simulink library "cntrlPosNdi_lib"  (R2018b)
settings: Solver=VariableStepAuto  StartTime=0.0  StopTime=10.0  RelTol=1e-3
undefined symbols (not defined in the file or in its folder): DiscIntNeverNeededParam, psc
libraries: filters_lib x3, simulink x2, $bdroot x2, stick_lib x1
settings Model: Creator=Ybeyer  LastModifiedBy=yannic
settings SFSimCC: SimUseLocalCustomCode=off
settings RTWCC: RTWUseLocalCustomCode=off
settings CodeAppCC: StateflowObjectComments=on

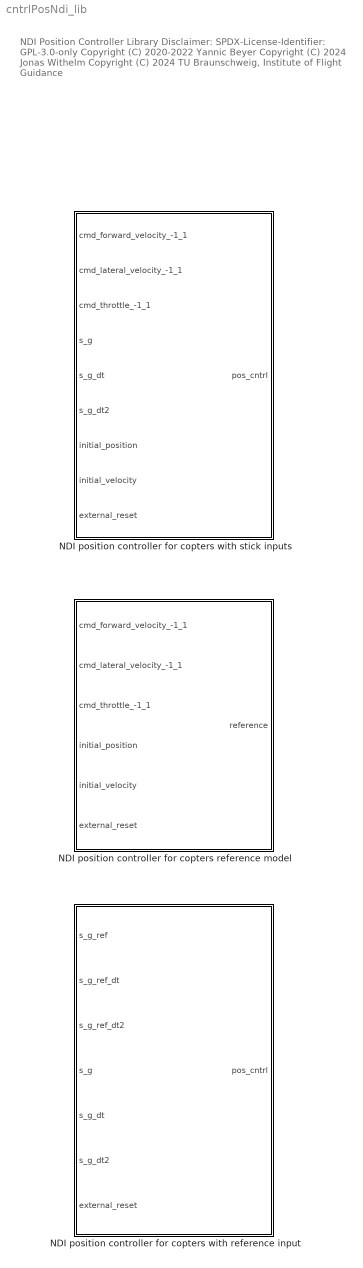
== system cntrlPosNdi_lib ==
  note: NDI Position Controller Library
      |
      | Disclaimer:
      | SPDX-License-Identifier: GPL-3.0-only
      |
      | Copyright (C) 2020-2022 Yannic Beyer
      | Copyright (C) 2024 Jonas Withelm
      | Copyright (C) 2024 TU Braunschweig, Institute of Flight Guidance
  NDI position controller for copters reference model : Subsystem  mask{psc=psc, is_enable_checked=off, states_when_enabling=held}
      mask prompts: psc "position controller parameters struct, see cntrlPosIndi_params_default"; is_enable_checked "Activate "Enabled Subsystem""; states_when_enabling "States when enabling:"
      mask init:
      | cntrlBlockInit(is_enable_checked,states_when_enabling);
      mask TypeOptions states_when_enabling: held | reset
      mask DialogControl DescGroupVar Prompt: NDI position controller for copters reference model
      mask DialogControl DescTextVar Prompt: The commanded velocity is filtered and reference signals are generated.
  NDI position controller for copters with reference input : Subsystem  mask{psc=psc, T_inner_loop=0.1, is_enable_checked=off, states_when_enabling=held, mask_expr_handling_config=default}
      mask prompts: psc "Position controller parameters struct, see cntrlPosIndi_params_default"; T_inner_loop "Inner loop time constant, in s"; is_enable_checked "Activate "Enabled Subsystem""; states_when_enabling "States when enabling:"
      mask init:
      | cntrlBlockInit(is_enable_checked,states_when_enabling);
      | 
      | maskExprHandling(gcbh, mask_expr_handling_config);
      mask TypeOptions states_when_enabling: held | reset
      mask TypeOptions mask_expr_handling_config: default | passthrough (tunable)
      mask DialogControl DescGroupVar Prompt: NDI position controller cascade with reference inputs
      mask DialogControl DescTextVar Prompt: The controller takes reference signals as input and the control error is converted into desired accerlations.
      mask DialogControl CodeGenerationSettings Prompt: Code Generation Settings
      mask DialogControl maskExprHandlingText Prompt: Mask expression handling
      mask DialogControl maskExprHandlingReadme Prompt: README
      mask DialogControl maskExprHandlingReadme Tooltip: https://github.com/iff-gsc/m-Utils/tree/main/simulink/mask_expression_handling/README.md
      mask DialogControl maskExprHandlingReadme Callback: web('https://github.com/iff-gsc/m-Utils/tree/main/simulink/mask_expression_handling/README.md','-browser')
  NDI position controller for copters with stick inputs : Subsystem  mask{psc=psc, T_inner_loop=0.1, is_enable_checked=off, states_when_enabling=held}
      mask prompts: psc "position controller parameters struct, see cntrlPosIndi_params_default"; T_inner_loop "inner loop time constant, in s"; is_enable_checked "Activate "Enabled Subsystem""; states_when_enabling "States when enabling:"
      mask init:
      | cntrlBlockInit(is_enable_checked,states_when_enabling);
      mask TypeOptions states_when_enabling: held | reset
      mask DialogControl DescGroupVar Prompt: NDI Position controller cascade
      mask DialogControl DescTextVar Prompt: The commanded velocity is filtered and the control error is converted into desired accerlations.

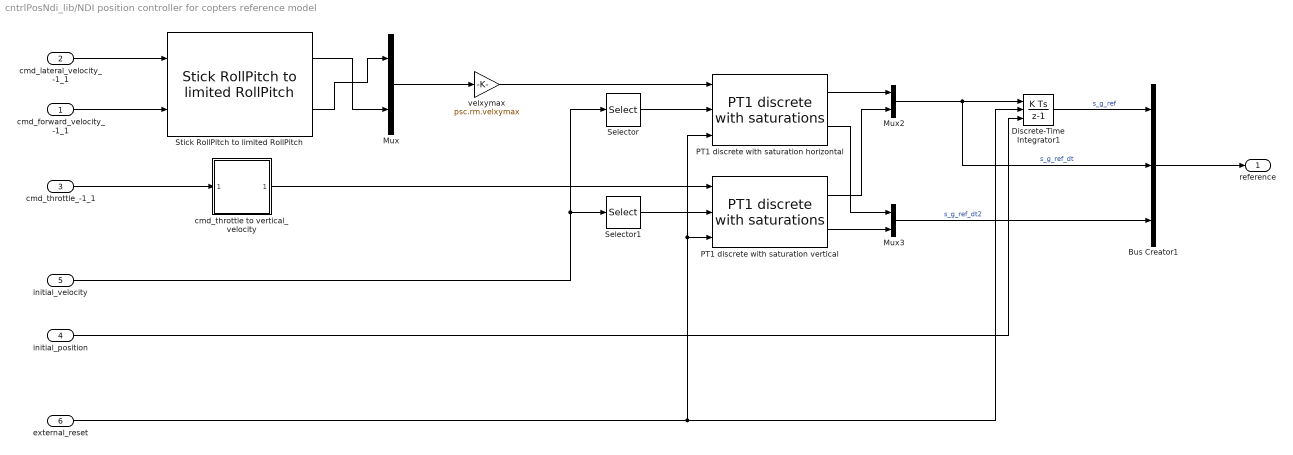
== system cntrlPosNdi_lib/NDI position controller for copters reference model ==
  cmd_forward_velocity_-1_1 : Inport
  cmd_lateral_velocity_-1_1 : Inport  Port=2
  cmd_throttle_-1_1 : Inport  Port=3
  initial_position : Inport  Port=4
  initial_velocity : Inport  Port=5
  external_reset : Inport  Port=6
  Bus Creator1 : BusCreator  Inputs=3
  Discrete-Time Integrator1 : DiscreteIntegrator  ExternalReset=rising  InitialConditionSource=external  SampleTime=-1  ICPrevOutput=DiscIntNeverNeededParam  ICPrevScaledInput=DiscIntNeverNeededParam
  Mux : Mux  Inputs=2
  Mux2 : Mux  Inputs=2
  Mux3 : Mux  Inputs=2
  PT1 discrete with saturation horizontal : filters_lib/PT1 discrete with saturations  param_src=internal  T=psc.rm.veltc  x_max=inf  x_min=-inf  x_dt_max=psc.rm.accxymax  x_dt_min=-psc.rm.accxymax  y_0_src=external  x_init=0  is_y_dt_checked=on  is_external_reset_checked=on  mask_expr_handling_config=passthrough (tunable)
      settings: SourceProductName=LADAC
  PT1 discrete with saturation vertical : filters_lib/PT1 discrete with saturations  param_src=internal  T=psc.rm.veltc  x_max=inf  x_min=-inf  x_dt_max=psc.rm.accdmax  x_dt_min=-psc.rm.accumax  y_0_src=external  x_init=0  is_y_dt_checked=on  is_external_reset_checked=on  mask_expr_handling_config=passthrough (tunable)
      settings: SourceProductName=LADAC
  Selector : Selector  InputPortWidth=3  IndexOptions=Index vector (dialog)  Indices=[1 2]  OutputSizes=1
  Selector1 : Selector  InputPortWidth=3  IndexOptions=Index vector (dialog)  Indices=[3]  OutputSizes=1
  Stick RollPitch to limited RollPitch : stick_lib/Stick RollPitch to limited RollPitch  limiting_mode=1
      settings: SourceProductName=LADAC
  cmd_throttle to vertical_velocity : Subsystem  mask(Throttle command to vertical velocity){veldmax=psc.rm.veldmax, velumax=psc.rm.velumax}
      mask help: Translates a throttle command [-1, 0, 1] to [veldmax, 0, -velumax]. A 1-D Lookup-Table would do the same job, but is not compatible with tunable parameter code generation when the array is defined in the parameter field (square bracket [] restriction).
  velxymax : Gain  Gain=psc.rm.velxymax
  reference : Outport
  wires:
  cmd_forward_velocity_-1_1/1 -> Stick RollPitch to limited RollPitch/2
  cmd_lateral_velocity_-1_1/1 -> Stick RollPitch to limited RollPitch/1
  Mux/1 -> velxymax/1
  cmd_throttle_-1_1/1 -> cmd_throttle to vertical_velocity/1(cmd_throttle)
  Stick RollPitch to limited RollPitch/1 -> Mux/2
  Stick RollPitch to limited RollPitch/2 -> Mux/1
  PT1 discrete with saturation vertical/1 -> Mux2/2
  Selector1/1 -> PT1 discrete with saturation vertical/2
  Mux2/1 -> Bus Creator1/2, Discrete-Time Integrator1/1  "s_g_ref_dt"
  PT1 discrete with saturation horizontal/2 -> Mux3/1
  PT1 discrete with saturation horizontal/1 -> Mux2/1
  Mux3/1 -> Bus Creator1/3  "s_g_ref_dt2"
  velxymax/1 -> PT1 discrete with saturation horizontal/1
  Discrete-Time Integrator1/1 -> Bus Creator1/1  "s_g_ref"
  Bus Creator1/1 -> reference/1
  initial_velocity/1 -> Selector1/1, Selector/1
  cmd_throttle to vertical_velocity/1(vertical_velocity) -> PT1 discrete with saturation vertical/1
  Selector/1 -> PT1 discrete with saturation horizontal/2
  PT1 discrete with saturation vertical/2 -> Mux3/2
  initial_position/1 -> Discrete-Time Integrator1/3
  external_reset/1 -> PT1 discrete with saturation vertical/3, PT1 discrete with saturation horizontal/3, Discrete-Time Integrator1/2

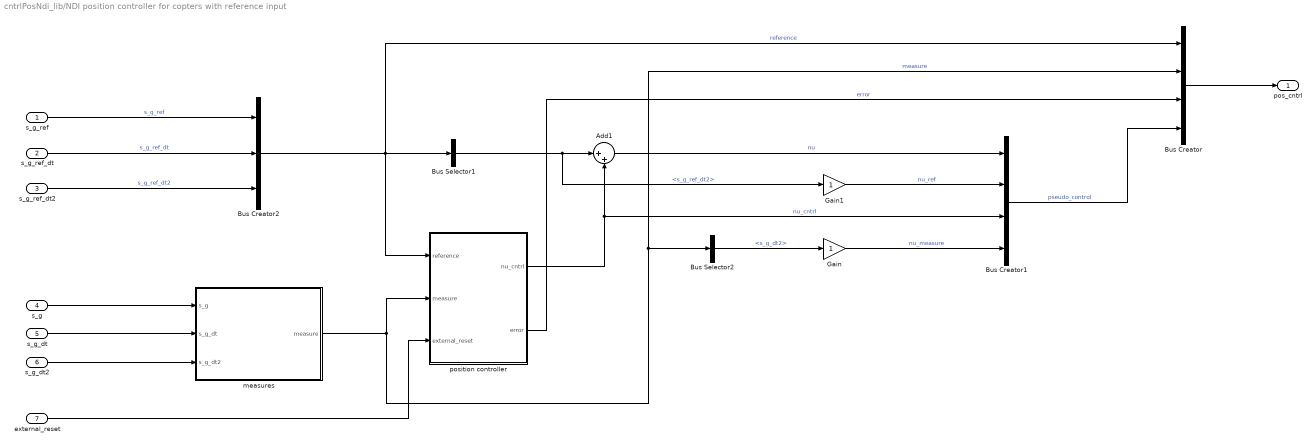
== system cntrlPosNdi_lib/NDI position controller for copters with reference input ==
  s_g_ref : Inport
  s_g_ref_dt : Inport  Port=2
  s_g_ref_dt2 : Inport  Port=3
  s_g : Inport  Port=4
  s_g_dt : Inport  Port=5
  s_g_dt2 : Inport  Port=6
  external_reset : Inport  Port=7
  Add1 : Sum  Inputs=|++
  Bus Creator : BusCreator  Inputs=4
  Bus Creator1 : BusCreator  Inputs=4
  Bus Creator2 : BusCreator  Inputs=3
  Bus Selector1 : BusSelector  OutputSignals=s_g_ref_dt2
  Bus Selector2 : BusSelector  OutputSignals=s_g_dt2
  Gain : Gain
  Gain1 : Gain
  measures : Subsystem
  position controller : Subsystem
  pos_cntrl : Outport
  wires:
  Bus Creator2/1 -> Bus Creator/1, position controller/1(reference), Bus Selector1/1  "reference"
  position controller/1(nu_cntrl) -> Add1/2, Bus Creator1/3  "nu_cntrl"
  Add1/1 -> Bus Creator1/1  "nu"
  s_g_dt2/1 -> measures/3(s_g_dt2)
  position controller/2(error) -> Bus Creator/3  "error"
  s_g/1 -> measures/1(s_g)
  s_g_dt/1 -> measures/2(s_g_dt)
  measures/1(measure) -> position controller/2(measure), Bus Selector2/1, Bus Creator/2  "measure"
  Bus Creator1/1 -> Bus Creator/4  "pseudo_control"
  Bus Creator/1 -> pos_cntrl/1
  Gain/1 -> Bus Creator1/4  "nu_measure"
  Bus Selector1/1 -> Gain1/1, Add1/1  "<s_g_ref_dt2>"
  Gain1/1 -> Bus Creator1/2  "nu_ref"
  s_g_ref/1 -> Bus Creator2/1  "s_g_ref"
  s_g_ref_dt/1 -> Bus Creator2/2  "s_g_ref_dt"
  s_g_ref_dt2/1 -> Bus Creator2/3  "s_g_ref_dt2"
  Bus Selector2/1 -> Gain/1  "<s_g_dt2>"
  external_reset/1 -> position controller/3(external_reset)

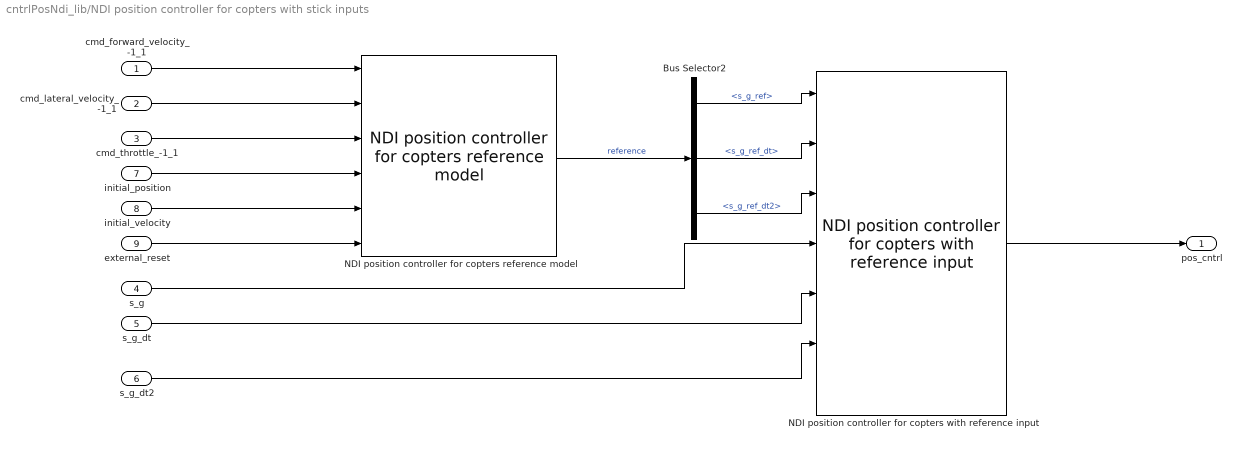
== system cntrlPosNdi_lib/NDI position controller for copters with stick inputs ==
  cmd_forward_velocity_-1_1 : Inport
  cmd_lateral_velocity_-1_1 : Inport  Port=2
  cmd_throttle_-1_1 : Inport  Port=3
  s_g : Inport  Port=4
  s_g_dt : Inport  Port=5
  s_g_dt2 : Inport  Port=6
  initial_position : Inport  Port=7
  initial_velocity : Inport  Port=8
  external_reset : Inport  Port=9
  Bus Selector2 : BusSelector  OutputSignals=s_g_ref,s_g_ref_dt,s_g_ref_dt2
  NDI position controller for copters reference model : $bdroot/NDI position controller for copters reference model  psc=psc  is_enable_checked=off  states_when_enabling=held
  NDI position controller for copters with reference input : $bdroot/NDI position controller for copters with reference input  psc=psc  T_inner_loop=T_inner_loop  is_enable_checked=off  states_when_enabling=held  mask_expr_handling_config=default
  pos_cntrl : Outport
  wires:
  cmd_forward_velocity_-1_1/1 -> NDI position controller for copters reference model/1
  initial_position/1 -> NDI position controller for copters reference model/4
  s_g_dt2/1 -> NDI position controller for copters with reference input/6
  s_g/1 -> NDI position controller for copters with reference input/4
  s_g_dt/1 -> NDI position controller for copters with reference input/5
  cmd_lateral_velocity_-1_1/1 -> NDI position controller for copters reference model/2
  cmd_throttle_-1_1/1 -> NDI position controller for copters reference model/3
  NDI position controller for copters reference model/1 -> Bus Selector2/1  "reference"
  Bus Selector2/1 -> NDI position controller for copters with reference input/1  "<s_g_ref>"
  Bus Selector2/2 -> NDI position controller for copters with reference input/2  "<s_g_ref_dt>"
  Bus Selector2/3 -> NDI position controller for copters with reference input/3  "<s_g_ref_dt2>"
  NDI position controller for copters with reference input/1 -> pos_cntrl/1
  external_reset/1 -> NDI position controller for copters reference model/6
  initial_velocity/1 -> NDI position controller for copters reference model/5

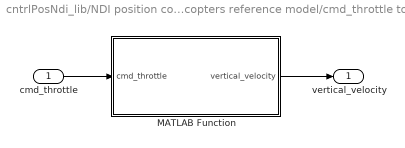
== system cntrlPosNdi_lib/NDI position controller for copters reference model/cmd_throttle to vertical_velocity ==
  cmd_throttle : Inport
  MATLAB Function : MATLAB Function  TreatAsAtomicUnit=on
  vertical_velocity : Outport
  wires:
  MATLAB Function/1(vertical_velocity) -> vertical_velocity/1
  cmd_throttle/1 -> MATLAB Function/1(cmd_throttle)

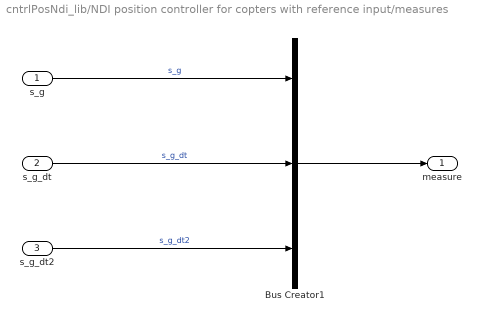
== system cntrlPosNdi_lib/NDI position controller for copters with reference input/measures ==
  s_g : Inport
  s_g_dt : Inport  Port=2
  s_g_dt2 : Inport  Port=3
  Bus Creator1 : BusCreator  Inputs=3
  measure : Outport
  wires:
  Bus Creator1/1 -> measure/1
  s_g_dt2/1 -> Bus Creator1/3  "s_g_dt2"
  s_g/1 -> Bus Creator1/1  "s_g"
  s_g_dt/1 -> Bus Creator1/2  "s_g_dt"

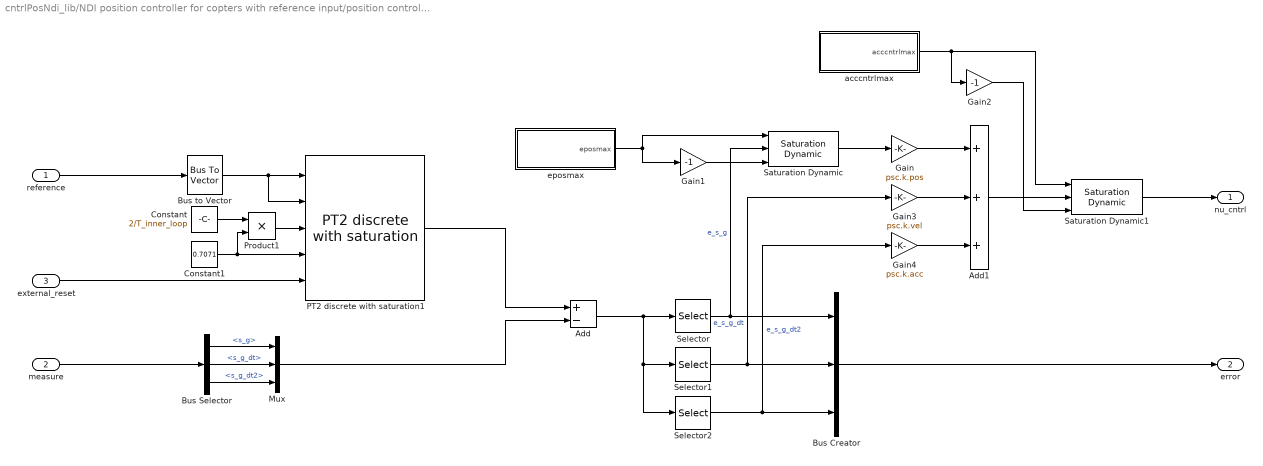
== system cntrlPosNdi_lib/NDI position controller for copters with reference input/position controller ==
  reference : Inport
  measure : Inport  Port=2
  external_reset : Inport  Port=3
  Add : Sum  Inputs=+-
  Add1 : Sum  Inputs=+++
  Bus Creator : BusCreator  Inputs=3
  Bus Selector : BusSelector  OutputSignals=s_g,s_g_dt,s_g_dt2
  Bus to Vector : BusToVector
  Constant : Constant  Value=2/T_inner_loop
  Constant1 : Constant  Value=0.7071
  Gain : Gain  Gain=psc.k.pos
  Gain1 : Gain  Gain=-1
  Gain2 : Gain  Gain=-1
  Gain3 : Gain  Gain=psc.k.vel
  Gain4 : Gain  Gain=psc.k.acc
  Mux : Mux  Inputs=3
  PT2 discrete with saturation1 : filters_lib/PT2 discrete with saturation  param_src=external  omega=1  d=0.7  x_max=inf  x_min=-inf  x_dt_max=inf  x_dt_min=-inf  x_dt2_max=inf  x_dt2_min=-inf  y_0_src=external  x_init=0  y_dt_0_src=internal  x_dt_init=0  is_y_dt_checked=off  is_y_dt2_checked=off  is_external_reset_checked=on  mask_expr_handling_config=default
      settings: SourceProductName=LADAC
  Product1 : Product
  Saturation Dynamic : simulink/Discontinuities/Saturation Dynamic  OutMin=[]  OutMax=[]  OutDataTypeStr=Inherit: Same as second input  OutDataType=fixdt(1, 16)  OutScaling=2^-10  DoSatur=off
  Saturation Dynamic1 : simulink/Discontinuities/Saturation Dynamic  OutMin=[]  OutMax=[]  OutDataTypeStr=Inherit: Same as second input  OutDataType=fixdt(1, 16)  OutScaling=2^-10  DoSatur=off
  Selector : Selector  InputPortWidth=9  IndexOptions=Index vector (dialog)  Indices=1:3  OutputSizes=1
  Selector1 : Selector  InputPortWidth=9  IndexOptions=Index vector (dialog)  Indices=4:6  OutputSizes=1
  Selector2 : Selector  InputPortWidth=9  IndexOptions=Index vector (dialog)  Indices=7:9  OutputSizes=1
  acccntrlmax : MATLAB Function  TreatAsAtomicUnit=on
  eposmax : MATLAB Function  TreatAsAtomicUnit=on
  nu_cntrl : Outport
  error : Outport  Port=2
  wires:
  reference/1 -> Bus to Vector/1
  Add/1 -> Selector2/1, Selector1/1, Selector/1
  Saturation Dynamic1/1 -> nu_cntrl/1
  Add1/1 -> Saturation Dynamic1/2
  measure/1 -> Bus Selector/1
  Mux/1 -> Add/2
  Bus Selector/3 -> Mux/3  "<s_g_dt2>"
  Bus Selector/2 -> Mux/2  "<s_g_dt>"
  Bus Selector/1 -> Mux/1  "<s_g>"
  Bus to Vector/1 -> PT2 discrete with saturation1/2, PT2 discrete with saturation1/1
  PT2 discrete with saturation1/1 -> Add/1
  Selector/1 -> Saturation Dynamic/2, Bus Creator/1  "e_s_g"
  Selector1/1 -> Bus Creator/2, Gain3/1  "e_s_g_dt"
  Selector2/1 -> Gain4/1, Bus Creator/3  "e_s_g_dt2"
  Bus Creator/1 -> error/1
  eposmax/1(eposmax) -> Saturation Dynamic/1, Gain1/1
  Gain1/1 -> Saturation Dynamic/3
  acccntrlmax/1(acccntrlmax) -> Saturation Dynamic1/1, Gain2/1
  Gain2/1 -> Saturation Dynamic1/3
  Gain/1 -> Add1/1
  Gain3/1 -> Add1/2
  Gain4/1 -> Add1/3
  Saturation Dynamic/1 -> Gain/1
  Constant/1 -> Product1/1
  Product1/1 -> PT2 discrete with saturation1/3
  Constant1/1 -> PT2 discrete with saturation1/4, Product1/2
  external_reset/1 -> PT2 discrete with saturation1/5

== matlab function cntrlPosNdi_lib/NDI position controller for copters with reference input/position controller/eposmax ==
  data: eposmax output; psc parameter
function eposmax = fcn(psc)
eposmax = abs( divideFinite( psc.k.vel * psc.rm.velxymax * 0.7, psc.k.pos ) );
end

== matlab function cntrlPosNdi_lib/NDI position controller for copters with reference input/position controller/acccntrlmax ==
  data: acccntrlmax output; psc parameter
function acccntrlmax = fcn(psc)
acccntrlmax = abs( 0.75 * psc.rm.accxymax );
end

== matlab function cntrlPosNdi_lib/NDI position controller for copters reference model/cmd_throttle to vertical_velocity/MATLAB Function ==
  data: cmd_throttle input; vertical_velocity output; veldmax parameter; velumax parameter
function vertical_velocity = fcn(cmd_throttle, veldmax, velumax)
    
    if cmd_throttle < 0
        vertical_velocity = -veldmax * cmd_throttle;
    else
        vertical_velocity = -velumax * cmd_throttle;
    end

end
